simulink model "microgrid"  (R2025b)
settings: Solver=daessc  StartTime=0.0  StopTime=600  FixedStep=1728.0  MaxStep=1728.0  RelTol=1e-3
PreLoadFcn:
  | microgrid_parameters
InitFcn:
  | microgrid_parameters
values from neighbouring files (symbols this model uses):
  PV = photovoltaic_parameters    [microgrid_parameters.m]
  URFC = urfc_parameters    [microgrid_parameters.m]
undefined symbols (not defined in the file or in its folder): BUS, URFC_TANK
libraries: fl_lib x28, nesl_utility x14, ee_lib x9, SignalEditorBlockLib x1
settings Model: Creator=michaelfsb  LastModifiedBy=DEVANG
settings DebuggingCC: IgnoredZcDiagnostic=error
settings RTWCC: GPUComputeCapability=3.5
settings SimscapeCC: SimscapeLogLimitData=off

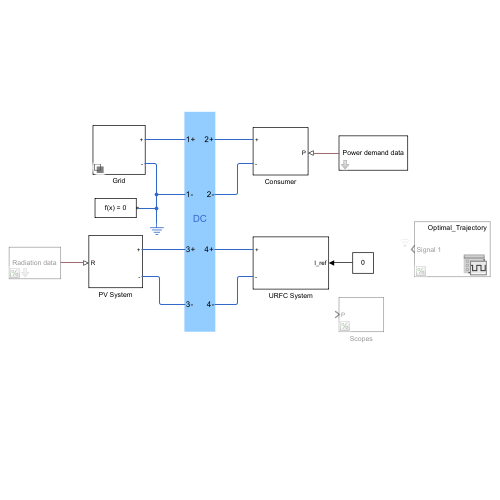
[thumbnail: Simulink's stored preview of the top-level diagram]
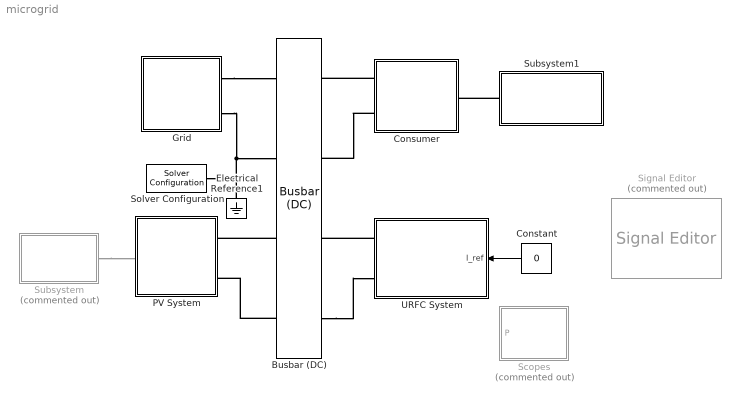
== system microgrid ==
  Busbar (DC) : ee_lib/Connectors & References/Busbar (DC)  n_nodes=ee.enum.connectors.busbar_number_of_connections.four  VRated=1e3 V  measurement_type=ee.enum.measurementType.instantaneous  averaging_period=1e-2 s  show_ps=ee.enum.connectors.busbar_measurement.false
      settings: InternalSimscapePortConfiguration="{\"Bottom\":[],\"Left\":[{\"id\":\"p1\",\"label\":\"1+\",\"type\":\"foundation.electrical.electrical\"},{\"id\":\"n1\",\"label\":\"1-\",\"type\":\"foundation.electrical.electrical\"},{\"id\":\"p3\",\"label\":\"3+\",\"type\":\"foundation.electrical.electrical\"},{\"id\":\"n3\",\"label\":\"3-\",\"type\":\"foundation.electrical.electrical\"}],\"Right\":[{\"id\":\"p2\",\"label\":\"2+\",\"type\":\"foundation.electrical.electrical\"},{\"id\":\"n2\",\"label\":\"2-\",\"type\":\"foundation.electrical.electrical\"},{\"id\":\"p4\",\"label\":\"4+\",\"type\":\"foundation.electrical.electrical\"},{\"id\":\"n4\",\"label\":\"4-\",\"type\":\"foundation.electrical.electrical\"}],\"Top\":[]}"
  Constant : Constant  Value=0
  Consumer : Subsystem
  Electrical Reference1 : fl_lib/Electrical/Electrical Elements/Electrical Reference
  Grid : Subsystem  Variant=on  VariantControlMode=label  VariantControl=Grid  LabelModeActiveChoice=AC1
      settings: PortSchema="{\"entries\":[{\"content\":{\"sides\":[{\"content\":{},\"type\":\"ConnectorPlacement.EquallySpacedRectSide\",\"uuid\":\"7d3e1531-3ac3-48d1-8d53-8dc071a39518\"},{\"content\":{\"side\":\"RIGHT\"},\"type\":\"ConnectorPlacement.EquallySpacedRectSide\",\"uuid\":\"25b50bd9-2b9f-4527-8fc7-8205feed0a4d\"},{\"content\":{\"connectorIds\":[\"LConn1\",\"LConn2\"],\"side\":\"TOP\"},\"type\":\"ConnectorPlacement.EquallySpacedRectSide\",\"uuid\":\"ec9d499b-92d3-45f6-91a8-3c7a2a7323b8\"}]},\"type\":\"ConnectorPlacement.EquallySpacedConnector\",\"uuid\":\"21f9d016-eefb-40e7-aeda-3b0d2900fe93\"}],\"packageUris\":[\"http://schema.mathworks.com/mf0/Connector/R2020b\"],\"version\":\"1.0\"}"
  PV System : Subsystem
      settings: PortSchema="{\"entries\":[{\"content\":{\"sides\":[{\"content\":{},\"type\":\"ConnectorPlacement.EquallySpacedRectSide\",\"uuid\":\"b223c642-574d-498e-9628-4dce2dfe786d\"},{\"content\":{\"side\":\"RIGHT\"},\"type\":\"ConnectorPlacement.EquallySpacedRectSide\",\"uuid\":\"c960ad2e-8659-4c85-9aee-0bfb29cbdae9\"},{\"content\":{\"connectorIds\":[\"LConn1\",\"LConn2\"],\"side\":\"TOP\"},\"type\":\"ConnectorPlacement.EquallySpacedRectSide\",\"uuid\":\"3aea4236-f32b-4c02-92e6-11ca7609eeb0\"},{\"content\":{\"connectorIds\":[\"RConn1\"],\"side\":\"BOTTOM\"},\"type\":\"ConnectorPlacement.EquallySpacedRectSide\",\"uuid\":\"59a771e4-e218-45af-8738-bea5dfc08a6d\"}]},\"type\":\"ConnectorPlacement.EquallySpacedConnector\",\"uuid\":\"f3a4f2e2-ab14-400c-a1b0-7ee7894a4fc3\"}],\"packageUris\":[\"http://schema.mathworks.com/mf0/Connector/R2020b\"],\"version\":\"1.0\"}"
  Scopes : Subsystem  Commented=on
  Signal Editor : SignalEditorBlockLib/Signal Editor  Commented=on  FileName=op_mode_siginal.mat  ActiveScenario=Optimal_Trajectory  ActiveSignal=i_el_ref  IsBus=off  OutputBusObjectStr=Bus: BusObject  SampleTime=0  ZeroCross=off  OutputAfterFinalValue=Setting to zero  Unit=inherit  PreserveSignalName=on  ApplySigPropsToAllScenarios=off  ApplySigPropsToAllSignals=on  SignalPropertySource=Dialog parameters
  Solver Configuration : nesl_utility/Solver Configuration  PhysicalDomain=network_engine_domain  SubClassName=solver  LeftPortType=input  RightPortType=generic  Tones=[]  Harmonics=[]  SimulateNoise=off  Profile=off  UseLocalSampling=off  EnableSwitchedLinearOptims=on  FrequencyDomain=off  UseCCode=off  RelTol=0.001  AbsTol=0.001  MinStep=1e-09  ToWorkspace=off  RevertToSquareIcSolve=off  NumHomotopyIterations=100  PhasorMode=off  PhasorModeNumHarmonics=1  ConsistencySolver=NEWTON_XTOL_AFTER_FTOL  IndexReductionMethod=DerivativeReplacement  DoDC=off  ResidualTolerance=1e-09  ConsistencyTolSource=GLOBAL  ConsistencyAbsTol=0.001  ConsistencyRelTol=0.001  ConsistencyTolFactor=0.001  UseLocalSolver=on  LocalSolverChoice=NE_BACKWARD_EULER_ADVANCER  ResolveIndetEquations=on  FunctionEvalNumThread=1  LocalSolverSampleTime=1  DoFixedCost=on  MaxNonlinIter=3  MaxModeIter=2  ComputeImpulses=off  ImpulseIterations=2  LinearAlgebra=auto  LinearAlgebraNumThread=0  EquationFormulation=NE_TIME_EF  DelaysMemoryBudget=1024  AutomaticFiltering=on  FilteringTimeConstant=0.001  PartitionStorageMethod=AS_NEEDED  PartitionMemoryBudget=1024  PartitionMethod=ROBUST  MultibodyUseLocalSolver=off  MultibodyLocalSolverChoice=ODE1  MultibodyLocalSolverSampleTime=0.001
  Subsystem : Subsystem  Commented=on
      mask Display: disp('Radiation data');
  Subsystem1 : Subsystem
      mask Display: disp('Power demand data');
  URFC System : Subsystem
  wires:
  Constant/1 -> URFC System/1(I_ref)
  connections:
  Busbar (DC)/LConn3 -- PV System/LConn1
  Consumer/LConn1 -- Busbar (DC)/RConn1
  Busbar (DC)/LConn4 -- PV System/LConn2
  Consumer/LConn2 -- Busbar (DC)/RConn2
  URFC System/RConn1 -- Busbar (DC)/RConn3
  Busbar (DC)/RConn4 -- URFC System/RConn2
  Subsystem/RConn1 -- PV System/RConn1
  Subsystem1/RConn1 -- Consumer/RConn1
  Grid/LConn2 -- Solver Configuration/RConn1 -- Electrical Reference1/LConn1 -- Busbar (DC)/LConn2
  Grid/LConn1 -- Busbar (DC)/LConn1

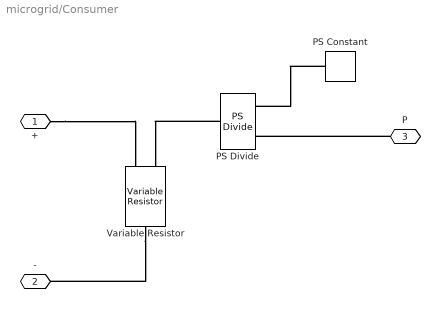
== system microgrid/Consumer ==
  PS Constant : fl_lib/Physical Signals/Sources/PS Constant  constant=BUS.Voltage^2 V^2
  PS Divide : fl_lib/Physical Signals/Functions/PS Divide
  Variable Resistor : fl_lib/Electrical/Electrical Elements/Variable Resistor  Rmin=0 Ohm  thermalEnable=false  thermal_mass=1 J/K  i_specify=off  i_priority=None  i=0 A  i_nominal_specify=off  i_nominal_value=1  i_nominal_unit=A  v_specify=off  v_priority=None  v=0 V  v_nominal_specify=off  v_nominal_value=1  v_nominal_unit=V  T_specify=off  T_priority=None  T=300 K  T_nominal_specify=off  T_nominal_value=1  T_nominal_unit=K
  + : PMIOPort  Side=Left
  - : PMIOPort  Port=2  Side=Left
  P : PMIOPort  Port=3  Side=Right
  connections:
  Variable Resistor/RConn1 -- -/RConn1
  PS Constant/RConn1 -- PS Divide/LConn1
  PS Divide/RConn1 -- Variable Resistor/LConn1
  +/RConn1 -- Variable Resistor/LConn2
  P/RConn1 -- PS Divide/LConn2

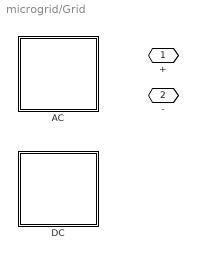
== system microgrid/Grid ==
  AC : Subsystem  VariantControl=Grid
      settings: PortSchema="{\"entries\":[{\"content\":{\"sides\":[{\"content\":{},\"type\":\"ConnectorPlacement.EquallySpacedRectSide\",\"uuid\":\"7d3e1531-3ac3-48d1-8d53-8dc071a39518\"},{\"content\":{\"side\":\"RIGHT\"},\"type\":\"ConnectorPlacement.EquallySpacedRectSide\",\"uuid\":\"25b50bd9-2b9f-4527-8fc7-8205feed0a4d\"},{\"content\":{\"connectorIds\":[\"LConn1\",\"LConn2\"],\"side\":\"TOP\"},\"type\":\"ConnectorPlacement.EquallySpacedRectSide\",\"uuid\":\"ec9d499b-92d3-45f6-91a8-3c7a2a7323b8\"}]},\"type\":\"ConnectorPlacement.EquallySpacedConnector\",\"uuid\":\"21f9d016-eefb-40e7-aeda-3b0d2900fe93\"}],\"packageUris\":[\"http://schema.mathworks.com/mf0/Connector/R2020b\"],\"version\":\"1.0\"}"
  DC : Subsystem  VariantControl=AC1
      settings: PortSchema="{\"entries\":[{\"content\":{\"sides\":[{\"content\":{},\"type\":\"ConnectorPlacement.EquallySpacedRectSide\",\"uuid\":\"7d3e1531-3ac3-48d1-8d53-8dc071a39518\"},{\"content\":{\"side\":\"RIGHT\"},\"type\":\"ConnectorPlacement.EquallySpacedRectSide\",\"uuid\":\"25b50bd9-2b9f-4527-8fc7-8205feed0a4d\"},{\"content\":{\"connectorIds\":[\"LConn1\",\"LConn2\"],\"side\":\"TOP\"},\"type\":\"ConnectorPlacement.EquallySpacedRectSide\",\"uuid\":\"ec9d499b-92d3-45f6-91a8-3c7a2a7323b8\"}]},\"type\":\"ConnectorPlacement.EquallySpacedConnector\",\"uuid\":\"21f9d016-eefb-40e7-aeda-3b0d2900fe93\"}],\"packageUris\":[\"http://schema.mathworks.com/mf0/Connector/R2020b\"],\"version\":\"1.0\"}"
  + : PMIOPort  Side=Left
  - : PMIOPort  Port=2  Side=Left

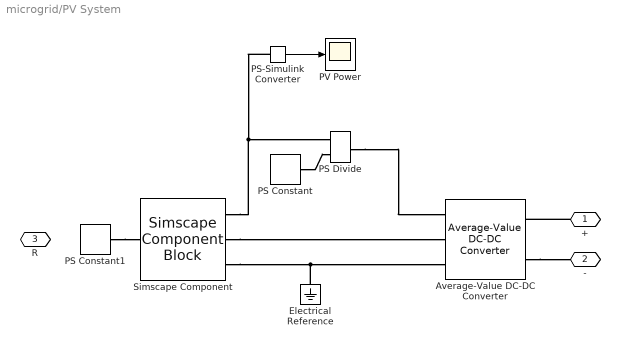
== system microgrid/PV System ==
  Average-Value DC-DC Converter : ee_lib/Semiconductors & Converters/Converters/Average-Value DC-DC Converter  implementation_option=ee.enum.converters.implementation.behavioral  converter_type=ee.enum.converters.dcdctype.boost  control_option=ee.enum.converters.controlinput.current  efficiency_option=ee.enum.converters.efficiency.constant  efficiency_fixed=100  i_vec=[0, 2, 5] A  efficiency_vec=[90, 95, 98]  Lf=1e-6 H  Rl=0 Ohm  Cf=1e-7 F  Rc=1e-6 Ohm  iL_specify=off  iL_priority=High  iL=0 A  iL_nominal_specify=off  iL_nominal_value=1  iL_nominal_unit=A  vc_specify=off  vc_priority=High  vc=0 V  vc_nominal_specify=off  vc_nominal_value=1  vc_nominal_unit=V
      settings: InternalSimscapePortConfiguration="{\"Bottom\":[],\"Left\":[{\"id\":\"Iref\",\"label\":\"Iref\",\"type\":\"input\"},{\"id\":\"p1\",\"label\":\"1+\",\"type\":\"foundation.electrical.electrical\"},{\"id\":\"n1\",\"label\":\"1-\",\"type\":\"foundation.electrical.electrical\"}],\"Right\":[{\"id\":\"p2\",\"label\":\"2+\",\"type\":\"foundation.electrical.electrical\"},{\"id\":\"n2\",\"label\":\"2-\",\"type\":\"foundation.electrical.electrical\"}],\"Top\":[]}"
  Electrical Reference : fl_lib/Electrical/Electrical Elements/Electrical Reference
  PS Constant : fl_lib/Physical Signals/Sources/PS Constant  constant=BUS.Voltage V
  PS Constant1 : fl_lib/Physical Signals/Sources/PS Constant  constant=0.5
  PS Divide : fl_lib/Physical Signals/Functions/PS Divide
  PS-Simulink Converter : nesl_utility/PS-Simulink Converter  PhysicalDomain=network_engine_domain  SubClassName=ps_output  LeftPortType=input  RightPortType=output  PseudoPeriodic=off  Frequencies=[]  VectorFormat=inherit  Unit=W  AffineConversion=off
  PV Power : Scope
      settings: ActiveDisplayYMinimum=2487.8736060654028  ActiveDisplayYMaximum=4487.8736060654028  DataLoggingVariableName=ScopeData4
  Simscape Component : SimscapeComponentBlock  SourceFile=pv_panel  ComponentPath=pv_panel  ComponentVariants="[\"pv_panel\"]"  ComponentVariantNames="[\"pv_panel\"]"  ClassName=pv_panel  SchemaVersion=1  Nps=PV.N_ps  Nss=PV.N_ss  T=PV.T_ps K  Tr=PV.Tr K  Isc=PV.Isc A  Kl=PV.Kl A/K  Ior=PV.Ior A  Ego=PV.Ego V  A=PV.A  v_specify=off  v_priority=None  v=0 V  v_nominal_specify=off  v_nominal_value=1  v_nominal_unit=V  i_specify=off  i_priority=None  i=0 A  i_nominal_specify=off  i_nominal_value=1  i_nominal_unit=A
      settings: CopyFcn=simscape.sscblock.internal.componentBlockCallback(gcbh,'COPY')  PreCopyFcn=simscape.sscblock.internal.componentBlockCallback(gcbh,'PRECOPY')  PreDeleteFcn=simscape.sscblock.internal.componentBlockCallback(gcbh,'PREDELETE')  InternalSimscapePortConfiguration="{\"Bottom\":[],\"Left\":[{\"id\":\"lambda\",\"label\":\"R\",\"type\":\"input\"}],\"Right\":[{\"id\":\"p_mppt\",\"label\":\"p\",\"type\":\"output\"},{\"id\":\"p\",\"label\":\"+\",\"type\":\"foundation.electrical.electrical\"},{\"id\":\"n\",\"label\":\"-\",\"type\":\"foundation.electrical.electrical\"}],\"Top\":[]}"
      mask Type: pv_panel
  + : PMIOPort  Side=Left
  - : PMIOPort  Port=2  Side=Left
  R : PMIOPort  Port=3  Side=Right
  wires:
  PS-Simulink Converter/1 -> PV Power/1
  connections:
  Electrical Reference/LConn1 -- Average-Value DC-DC Converter/LConn3 -- Simscape Component/RConn3
  Simscape Component/RConn2 -- Average-Value DC-DC Converter/LConn2
  PS Constant/RConn1 -- PS Divide/LConn2
  Simscape Component/RConn1 -- PS-Simulink Converter/LConn1 -- PS Divide/LConn1
  PS Divide/RConn1 -- Average-Value DC-DC Converter/LConn1
  +/RConn1 -- Average-Value DC-DC Converter/RConn1
  Average-Value DC-DC Converter/RConn2 -- -/RConn1
  PS Constant1/RConn1 -- Simscape Component/LConn1

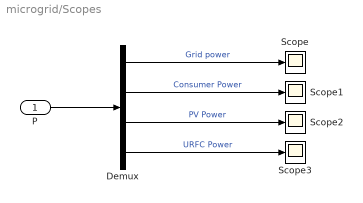
== system microgrid/Scopes ==
  P : Inport
  Demux : Demux
  Scope{,1..3} (4 alike) : Scope
      Scope2 settings: DataLoggingVariableName=ScopeData2
      Scope3 settings: DataLoggingVariableName=ScopeData3
  wires:
  P/1 -> Demux/1
  Demux/1 -> Scope/1  "Grid power"
  Demux/4 -> Scope3/1  "URFC Power"
  Demux/2 -> Scope1/1  "Consumer Power"
  Demux/3 -> Scope2/1  "PV Power"

== system microgrid/Subsystem ==
  PS Lookup Table (1D) : fl_lib/Physical Signals/Lookup Tables/PS Lookup Table (1D)  x=radiation.time  f=radiation.data  interp_method=simscape.enum.interpolation.linear  extrap_method=simscape.enum.extrapolation.linear
  PS Ramp : fl_lib/Physical Signals/Sources/PS Ramp  slope=1 1/s  start_time=0 s  initial_output=0  ZeroCross=true
  Conn1 : PMIOPort  Side=Right
  connections:
  PS Lookup Table (1D)/RConn1 -- Conn1/RConn1
  PS Ramp/RConn1 -- PS Lookup Table (1D)/LConn1

== system microgrid/Subsystem1 ==
  PS Lookup Table (1D)1 : fl_lib/Physical Signals/Lookup Tables/PS Lookup Table (1D)  x=power_demand.time  f=power_demand.data W  interp_method=simscape.enum.interpolation.linear  extrap_method=simscape.enum.extrapolation.linear
  PS Ramp1 : fl_lib/Physical Signals/Sources/PS Ramp  slope=1 1/s  start_time=0 s  initial_output=0  ZeroCross=true
  Conn1 : PMIOPort  Side=Right
  connections:
  PS Lookup Table (1D)1/RConn1 -- Conn1/RConn1
  PS Ramp1/RConn1 -- PS Lookup Table (1D)1/LConn1

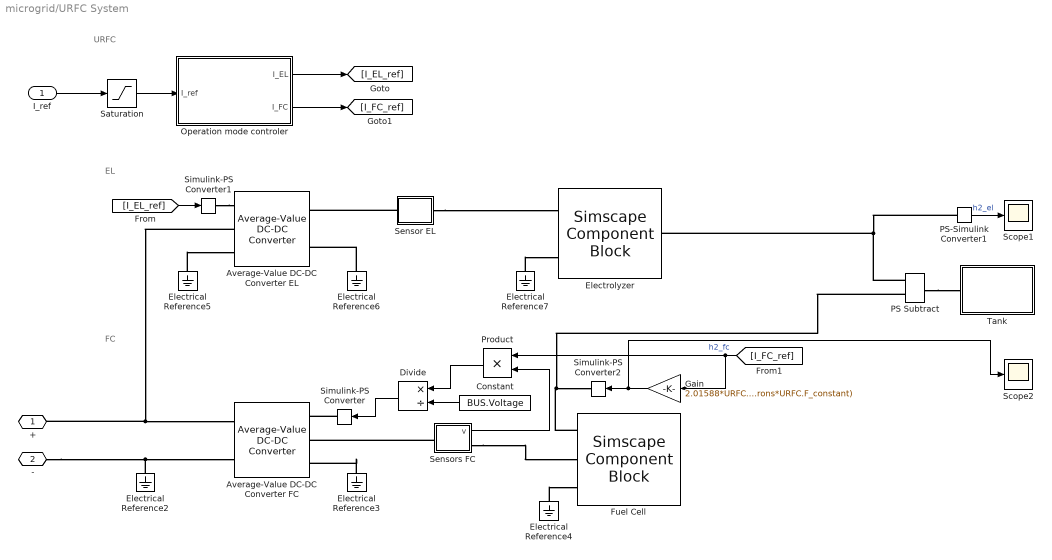
== system microgrid/URFC System ==
  note: URFC
  note: FC
  note: EL
  I_ref : Inport
  Average-Value DC-DC Converter EL : ee_lib/Semiconductors & Converters/Converters/Average-Value DC-DC Converter  implementation_option=ee.enum.converters.implementation.behavioral  converter_type=ee.enum.converters.dcdctype.buck  control_option=ee.enum.converters.controlinput.current  efficiency_option=ee.enum.converters.efficiency.tabulated  efficiency_fixed=100  i_vec=[0, 100, 200] A  efficiency_vec=[90, 95, 98]  Lf=1e-6 H  Rl=0 Ohm  Cf=1e-7 F  Rc=1e-6 Ohm  iL_specify=off  iL_priority=High  iL=0 A  iL_nominal_specify=off  iL_nominal_value=1  iL_nominal_unit=A  vc_specify=off  vc_priority=High  vc=0 V  vc_nominal_specify=off  vc_nominal_value=1  vc_nominal_unit=V
      settings: InternalSimscapePortConfiguration="{\"Bottom\":[],\"Left\":[{\"id\":\"Iref\",\"label\":\"Iref\",\"type\":\"input\"},{\"id\":\"p1\",\"label\":\"1+\",\"type\":\"foundation.electrical.electrical\"},{\"id\":\"n1\",\"label\":\"1-\",\"type\":\"foundation.electrical.electrical\"}],\"Right\":[{\"id\":\"p2\",\"label\":\"2+\",\"type\":\"foundation.electrical.electrical\"},{\"id\":\"n2\",\"label\":\"2-\",\"type\":\"foundation.electrical.electrical\"}],\"Top\":[]}"
  Average-Value DC-DC Converter FC : ee_lib/Semiconductors & Converters/Converters/Average-Value DC-DC Converter  implementation_option=ee.enum.converters.implementation.behavioral  converter_type=ee.enum.converters.dcdctype.boost  control_option=ee.enum.converters.controlinput.current  efficiency_option=ee.enum.converters.efficiency.constant  efficiency_fixed=100  i_vec=[0, 0.75, 2] A  efficiency_vec=[90, 95, 98]  Lf=1e-6 H  Rl=0 Ohm  Cf=1e-7 F  Rc=1e-6 Ohm  iL_specify=off  iL_priority=High  iL=0 A  iL_nominal_specify=off  iL_nominal_value=1  iL_nominal_unit=A  vc_specify=off  vc_priority=High  vc=0 V  vc_nominal_specify=off  vc_nominal_value=1  vc_nominal_unit=V
      settings: InternalSimscapePortConfiguration="{\"Bottom\":[],\"Left\":[{\"id\":\"Iref\",\"label\":\"Iref\",\"type\":\"input\"},{\"id\":\"p1\",\"label\":\"1+\",\"type\":\"foundation.electrical.electrical\"},{\"id\":\"n1\",\"label\":\"1-\",\"type\":\"foundation.electrical.electrical\"}],\"Right\":[{\"id\":\"p2\",\"label\":\"2+\",\"type\":\"foundation.electrical.electrical\"},{\"id\":\"n2\",\"label\":\"2-\",\"type\":\"foundation.electrical.electrical\"}],\"Top\":[]}"
  Constant : Constant  Value=BUS.Voltage
  Divide : Product  Inputs=*/
  Electrical Reference{2..7} (6 alike) : fl_lib/Electrical/Electrical Elements/Electrical Reference
  Electrolyzer : SimscapeComponentBlock  SourceFile=urfc_electrolyzer  ComponentPath=urfc_electrolyzer  ComponentVariants="[\"urfc_electrolyzer\"]"  ComponentVariantNames="[\"urfc_electrolyzer\"]"  ClassName=urfc_electrolyzer  SchemaVersion=1  N_cells=URFC.N_cells  A_cell=URFC.A_cell cm^2  E_rev_0=URFC.E_rev_0 V  I_loss_internal=URFC.I_loss_internal A/cm^2  I_o_anode=URFC.I_o_anode A/cm^2  I_o_cathode=URFC.I_o_cathode A/cm^2  R_ion=URFC.R_ion Ohm*cm^2  R_CR=URFC.R_CR Ohm*cm^2  R_elect=URFC.R_elect Ohm*cm^2  I_limit_anode=URFC.I_limit_anode A/cm^2  I_limit_cathode=URFC.I_limit_cathode A/cm^2  A_anodo=URFC.K_anodo V  A_catodo=URFC.K_catodo V  T=URFC.T K  R_gas=URFC.R_gas J/(K*mol)  F_constant=URFC.F_constant C/mol  n_electrons=URFC.n_electrons  i_specify=off  i_priority=None  i=0 A  i_nominal_specify=off  i_nominal_value=1  i_nominal_unit=A  v_specify=off  v_priority=None  v=0 V  v_nominal_specify=off  v_nominal_value=1  v_nominal_unit=V
      settings: CopyFcn=simscape.sscblock.internal.componentBlockCallback(gcbh,'COPY')  PreCopyFcn=simscape.sscblock.internal.componentBlockCallback(gcbh,'PRECOPY')  PreDeleteFcn=simscape.sscblock.internal.componentBlockCallback(gcbh,'PREDELETE')  LogSimulationData=on  InternalSimscapePortConfiguration="{\"Bottom\":[],\"Left\":[{\"id\":\"p\",\"label\":\"+\",\"type\":\"foundation.electrical.electrical\"},{\"id\":\"n\",\"label\":\"-\",\"type\":\"foundation.electrical.electrical\"}],\"Right\":[{\"id\":\"h2\",\"label\":\"H2\",\"type\":\"output\"}],\"Top\":[]}"
      mask Type: Electrolyzer mode model of a URFC
  Fuel Cell : SimscapeComponentBlock  SourceFile=urfc_fuel_cell  ComponentPath=urfc_fuel_cell  ComponentVariants="[\"urfc_fuel_cell\"]"  ComponentVariantNames="[\"urfc_fuel_cell\"]"  ClassName=urfc_fuel_cell  SchemaVersion=1  N_cells=URFC.N_cells  A_cell=URFC.A_cell cm^2  E_rev_0=1.23 V  I_loss_internal=URFC.I_loss_internal A/cm^2  I_o_anode=URFC.I_o_anode A/cm^2  I_o_cathode=URFC.I_o_cathode A/cm^2  R_ion=URFC.R_ion Ohm*cm^2  R_CR=URFC.R_CR Ohm*cm^2  R_elect=URFC.R_elect Ohm*cm^2  I_limit_anode=URFC.I_limit_anode A/cm^2  I_limit_cathode=URFC.I_limit_cathode A/cm^2  A_anodo=URFC.K_anodo V  A_catodo=URFC.K_catodo V  T=URFC.T K  R_gas=URFC.R_gas J/(K*mol)  F_constant=URFC.F_constant C/mol  n_electrons=2  i_specify=off  i_priority=None  i=0 A  i_nominal_specify=off  i_nominal_value=1  i_nominal_unit=A  v_specify=off  v_priority=None  v=0 V  v_nominal_specify=off  v_nominal_value=1  v_nominal_unit=V
      settings: CopyFcn=simscape.sscblock.internal.componentBlockCallback(gcbh,'COPY')  PreCopyFcn=simscape.sscblock.internal.componentBlockCallback(gcbh,'PRECOPY')  PreDeleteFcn=simscape.sscblock.internal.componentBlockCallback(gcbh,'PREDELETE')  LogSimulationData=on  InternalSimscapePortConfiguration="{\"Bottom\":[],\"Left\":[{\"id\":\"h2_in\",\"label\":\"H2_in\",\"type\":\"input\"},{\"id\":\"p\",\"label\":\"+\",\"type\":\"foundation.electrical.electrical\"},{\"id\":\"n\",\"label\":\"-\",\"type\":\"foundation.electrical.electrical\"}],\"Right\":[],\"Top\":[]}"
      mask Type: Fuel Cell mode model of a URFC
  Gain : Gain  Gain=2.01588*URFC.N_cells/(URFC.n_electrons*URFC.F_constant)
  Operation mode controler : Stateflow chart  TreatAsAtomicUnit=on
  PS Subtract : fl_lib/Physical Signals/Functions/PS Subtract
  PS-Simulink Converter1 : nesl_utility/PS-Simulink Converter  PhysicalDomain=network_engine_domain  SubClassName=ps_output  LeftPortType=input  RightPortType=output  PseudoPeriodic=off  Frequencies=[]  VectorFormat=inherit  Unit=inherit  AffineConversion=off
  Product : Product
  Saturation : Saturate  UpperLimit=200  LowerLimit=-200
  Scope1 : Scope
      settings: ActiveDisplayYMinimum=-0.00418  ActiveDisplayYMaximum=0.03763
  Scope2 : Scope
      settings: ActiveDisplayYMinimum=-1  ActiveDisplayYMaximum=1  DataLoggingVariableName=ScopeData2
  Sensor EL : Subsystem
  Sensors FC : Subsystem
  Simulink-PS Converter : nesl_utility/Simulink-PS Converter  PhysicalDomain=network_engine_domain  SubClassName=ps_input  LeftPortType=input  RightPortType=output  PseudoPeriodic=off  Frequencies=[]  NoiseDistribution=none  NoiseParameters=[]  Unit=1  AffineConversion=off  FilteringAndDerivatives=provide  SimscapeFilterOrder=1  InputFilterTimeConstant=0.001  UdotUserProvided=0
  Simulink-PS Converter1 : nesl_utility/Simulink-PS Converter  PhysicalDomain=network_engine_domain  SubClassName=ps_input  LeftPortType=input  RightPortType=output  PseudoPeriodic=off  Frequencies=[]  NoiseDistribution=none  NoiseParameters=[]  Unit=1  AffineConversion=off  FilteringAndDerivatives=provide  SimscapeFilterOrder=1  InputFilterTimeConstant=0.001  UdotUserProvided=0
  Simulink-PS Converter2 : nesl_utility/Simulink-PS Converter  PhysicalDomain=network_engine_domain  SubClassName=ps_input  LeftPortType=input  RightPortType=output  PseudoPeriodic=off  Frequencies=[]  NoiseDistribution=none  NoiseParameters=[]  Unit=g/s  AffineConversion=off  FilteringAndDerivatives=provide  SimscapeFilterOrder=1  InputFilterTimeConstant=0.001  UdotUserProvided=0
  Tank : Subsystem
  + : PMIOPort  Side=Right
  - : PMIOPort  Port=2  Side=Right
  wires:
  Constant/1 -> Divide/2
  Product/1 -> Divide/1
  [I_FC_ref] -> Gain/1, Product/1
  Sensors FC/1(v) -> Product/2
  Divide/1 -> Simulink-PS Converter/1
  Saturation/1 -> Operation mode controler/1(I_ref)
  Operation mode controler/2(I_FC) -> [I_FC_ref]
  Operation mode controler/1(I_EL) -> [I_EL_ref]
  I_ref/1 -> Saturation/1
  [I_EL_ref] -> Simulink-PS Converter1/1
  Gain/1 -> Scope2/1, Simulink-PS Converter2/1  "h2_fc"
  PS-Simulink Converter1/1 -> Scope1/1  "h2_el"
  connections:
  Sensors FC/RConn1 -- Fuel Cell/LConn2
  PS-Simulink Converter1/LConn1 -- PS Subtract/LConn1 -- Electrolyzer/RConn1
  Electrical Reference5/LConn1 -- Average-Value DC-DC Converter EL/LConn3
  Simulink-PS Converter1/RConn1 -- Average-Value DC-DC Converter EL/LConn1
  Electrical Reference6/LConn1 -- Average-Value DC-DC Converter EL/RConn2
  Sensor EL/RConn1 -- Average-Value DC-DC Converter EL/RConn1
  Sensors FC/LConn1 -- Average-Value DC-DC Converter FC/LConn2
  Simulink-PS Converter/RConn1 -- Average-Value DC-DC Converter FC/LConn1
  Electrical Reference3/LConn1 -- Average-Value DC-DC Converter FC/LConn3
  Electrical Reference2/LConn1 -- -/RConn1 -- Average-Value DC-DC Converter FC/RConn2
  Average-Value DC-DC Converter EL/LConn2 -- +/RConn1 -- Average-Value DC-DC Converter FC/RConn1
  Electrical Reference4/LConn1 -- Fuel Cell/LConn3
  Sensor EL/LConn1 -- Electrolyzer/LConn1
  Electrical Reference7/LConn1 -- Electrolyzer/LConn2
  PS Subtract/RConn1 -- Tank/LConn1
  Fuel Cell/LConn1 -- PS Subtract/LConn2 -- Simulink-PS Converter2/RConn1

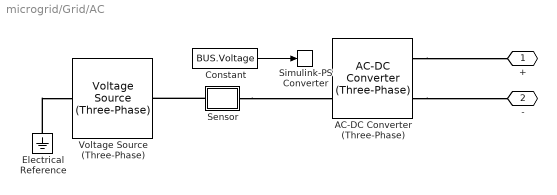
== system microgrid/Grid/AC ==
  AC-DC Converter (Three-Phase) : ee_lib/Semiconductors & Converters/Converters/AC-DC Converter (Three-Phase)  port_option=ee.enum.threePhasePort.composite  droop=0 V/A  Vdc_dynamics=ee.enum.converters.dynamics.no  tauVdc=0.02 s  Vdc_ini=100 V  FRated=60 Hz  Vline_rms_min=0.8*sqrt(3) * 100 / sqrt(2) V  tauVac=0.001 s  Vline_rms_ini=sqrt(3) * 100 / sqrt(2) V  Vang_ini=0 deg  power_dynamics=ee.enum.converters.powerDynamics.no  tauP=0.01 s  P_ini=1e3 W  gmin=1e-6 S
      settings: InternalSimscapePortConfiguration="{\"Bottom\":[],\"Left\":[{\"id\":\"Vref\",\"label\":\"Vref\",\"type\":\"input\"},{\"id\":\"N\",\"label\":\"~\",\"type\":\"foundation.electrical.three_phase\"}],\"Right\":[{\"id\":\"p\",\"label\":\"+\",\"type\":\"foundation.electrical.electrical\"},{\"id\":\"n\",\"label\":\"-\",\"type\":\"foundation.electrical.electrical\"}],\"Top\":[]}"
  Constant : Constant  Value=BUS.Voltage
  Electrical Reference : fl_lib/Electrical/Electrical Elements/Electrical Reference
  Sensor : Subsystem
      mask Display: disp('P');
  Simulink-PS Converter : nesl_utility/Simulink-PS Converter  PhysicalDomain=network_engine_domain  SubClassName=ps_input  LeftPortType=input  RightPortType=output  PseudoPeriodic=off  Frequencies=[]  NoiseDistribution=none  NoiseParameters=[]  Unit=V  AffineConversion=off  FilteringAndDerivatives=provide  SimscapeFilterOrder=1  InputFilterTimeConstant=0.001  UdotUserProvided=0
  Voltage Source (Three-Phase) : ee_lib/Sources/Voltage Source (Three-Phase)  vline_rms=sqrt(3) * 100 / sqrt(2) V  shift=0 deg  freq=60 Hz  impedance_option=1  SShortCircuit=1e6 A*V  XR=15  R=0.01 Ohm  L=3.97e-4 H  harmonic_option=0  harmonic_orders=[5, 7, 11, 13]  harmonic_ratios=[.1, .1, .1, .1]  G_parasitic=0 1/Ohm  I_specify=off  I_priority=None  I=[0, 0, 0] A  I_nominal_specify=off  I_nominal_unit=A  I_nominal_value=1
  + : PMIOPort  Side=Left
  - : PMIOPort  Port=2  Side=Left
  wires:
  Constant/1 -> Simulink-PS Converter/1
  connections:
  AC-DC Converter (Three-Phase)/RConn1 -- +/RConn1
  AC-DC Converter (Three-Phase)/RConn2 -- -/RConn1
  Sensor/RConn1 -- AC-DC Converter (Three-Phase)/LConn2
  Sensor/LConn1 -- Voltage Source (Three-Phase)/RConn1
  Electrical Reference/LConn1 -- Voltage Source (Three-Phase)/LConn1

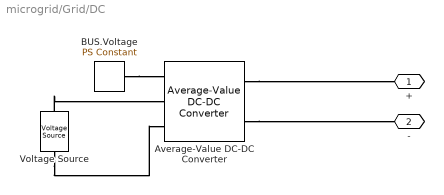
== system microgrid/Grid/DC ==
  Average-Value DC-DC Converter : ee_lib/Semiconductors & Converters/Converters/Average-Value DC-DC Converter  implementation_option=ee.enum.converters.implementation.behavioral  converter_type=ee.enum.converters.dcdctype.buck  control_option=ee.enum.converters.controlinput.voltage  efficiency_option=ee.enum.converters.efficiency.constant  efficiency_fixed=95  i_vec=[0, 2, 5] A  efficiency_vec=[90, 95, 98]  Lf=1e-6 H  Rl=0 Ohm  Cf=1e-7 F  Rc=1e-6 Ohm  iL_specify=off  iL_priority=High  iL=0 A  iL_nominal_specify=off  iL_nominal_value=1  iL_nominal_unit=A  vc_specify=off  vc_priority=High  vc=0 V  vc_nominal_specify=off  vc_nominal_value=1  vc_nominal_unit=V
      settings: InternalSimscapePortConfiguration="{\"Bottom\":[],\"Left\":[{\"id\":\"Vref\",\"label\":\"Vref\",\"type\":\"input\"},{\"id\":\"p1\",\"label\":\"1+\",\"type\":\"foundation.electrical.electrical\"},{\"id\":\"n1\",\"label\":\"1-\",\"type\":\"foundation.electrical.electrical\"}],\"Right\":[{\"id\":\"p2\",\"label\":\"2+\",\"type\":\"foundation.electrical.electrical\"},{\"id\":\"n2\",\"label\":\"2-\",\"type\":\"foundation.electrical.electrical\"}],\"Top\":[]}"
  BUS.Voltage : fl_lib/Physical Signals/Sources/PS Constant  constant=BUS.Voltage V
  Voltage Source : ee_lib/Sources/Voltage Source  dc_voltage=BUS.Voltage V  ac_voltage=0 V  ac_shift=0 rad  ac_frequency=60 Hz  noise_mode=ee.enum.sources.noise.Disabled  PSD=0 V^2/Hz  sample_time=1e-3 s  repeatability=ee.enum.sources.repeatability.NotRepeatable  user_seed=0  auto_seed=1129453067  i_specify=off  i_priority=None  i=0 A  i_nominal_specify=off  i_nominal_value=1  i_nominal_unit=A  v_specify=off  v_priority=None  v=0 V  v_nominal_specify=off  v_nominal_value=1  v_nominal_unit=V
  + : PMIOPort  Side=Left
  - : PMIOPort  Port=2  Side=Left
  connections:
  Voltage Source/LConn1 -- Average-Value DC-DC Converter/LConn2
  Voltage Source/RConn1 -- Average-Value DC-DC Converter/LConn3
  BUS.Voltage/RConn1 -- Average-Value DC-DC Converter/LConn1
  Average-Value DC-DC Converter/RConn1 -- +/RConn1
  Average-Value DC-DC Converter/RConn2 -- -/RConn1

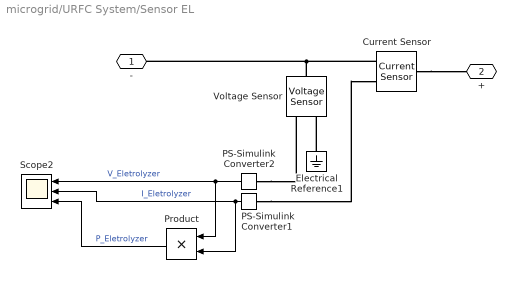
== system microgrid/URFC System/Sensor EL ==
  Current Sensor : fl_lib/Electrical/Electrical Sensors/Current Sensor
  Electrical Reference1 : fl_lib/Electrical/Electrical Elements/Electrical Reference
  PS-Simulink Converter1 : nesl_utility/PS-Simulink Converter  PhysicalDomain=network_engine_domain  SubClassName=ps_output  LeftPortType=input  RightPortType=output  PseudoPeriodic=off  Frequencies=[]  VectorFormat=inherit  Unit=inherit  AffineConversion=off
  PS-Simulink Converter2 : nesl_utility/PS-Simulink Converter  PhysicalDomain=network_engine_domain  SubClassName=ps_output  LeftPortType=input  RightPortType=output  PseudoPeriodic=off  Frequencies=[]  VectorFormat=inherit  Unit=inherit  AffineConversion=off
  Product : Product
  Scope2 : Scope  NumInputPorts=3
      settings: ActiveDisplayYMinimum=-52.2579  ActiveDisplayYMaximum=561.36199
  Voltage Sensor : fl_lib/Electrical/Electrical Sensors/Voltage Sensor
  - : PMIOPort  Side=Left
  + : PMIOPort  Port=2  Side=Right
  wires:
  PS-Simulink Converter2/1 -> Product/1, Scope2/1  "V_Eletrolyzer"
  PS-Simulink Converter1/1 -> Scope2/2, Product/2  "I_Eletrolyzer"
  Product/1 -> Scope2/3  "P_Eletrolyzer"
  connections:
  Current Sensor/LConn1 -- +/RConn1
  Electrical Reference1/LConn1 -- Voltage Sensor/RConn2
  PS-Simulink Converter2/LConn1 -- Voltage Sensor/RConn1
  Current Sensor/RConn2 -- Voltage Sensor/LConn1 -- -/RConn1
  PS-Simulink Converter1/LConn1 -- Current Sensor/RConn1

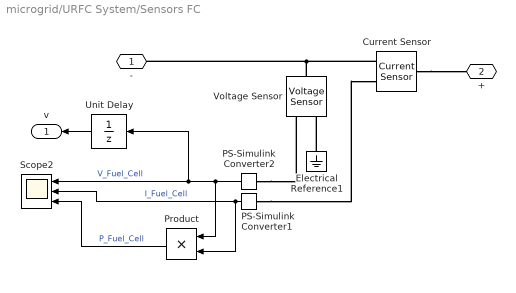
== system microgrid/URFC System/Sensors FC ==
  Current Sensor : fl_lib/Electrical/Electrical Sensors/Current Sensor
  Electrical Reference1 : fl_lib/Electrical/Electrical Elements/Electrical Reference
  PS-Simulink Converter1 : nesl_utility/PS-Simulink Converter  PhysicalDomain=network_engine_domain  SubClassName=ps_output  LeftPortType=input  RightPortType=output  PseudoPeriodic=off  Frequencies=[]  VectorFormat=inherit  Unit=inherit  AffineConversion=off
  PS-Simulink Converter2 : nesl_utility/PS-Simulink Converter  PhysicalDomain=network_engine_domain  SubClassName=ps_output  LeftPortType=input  RightPortType=output  PseudoPeriodic=off  Frequencies=[]  VectorFormat=inherit  Unit=inherit  AffineConversion=off
  Product : Product
  Scope2 : Scope  NumInputPorts=3
      settings: ActiveDisplayYMinimum=-52.2579  ActiveDisplayYMaximum=561.36199
  Unit Delay : UnitDelay  SampleTime=-1  HasFrameUpgradeWarning=on
  Voltage Sensor : fl_lib/Electrical/Electrical Sensors/Voltage Sensor
  - : PMIOPort  Side=Left
  + : PMIOPort  Port=2  Side=Right
  v : Outport
  wires:
  PS-Simulink Converter2/1 -> Product/1, Unit Delay/1, Scope2/1  "V_Fuel_Cell"
  PS-Simulink Converter1/1 -> Scope2/2, Product/2  "I_Fuel_Cell"
  Product/1 -> Scope2/3  "P_Fuel_Cell"
  Unit Delay/1 -> v/1
  connections:
  Current Sensor/LConn1 -- +/RConn1
  Electrical Reference1/LConn1 -- Voltage Sensor/RConn2
  PS-Simulink Converter2/LConn1 -- Voltage Sensor/RConn1
  Current Sensor/RConn2 -- -/RConn1 -- Voltage Sensor/LConn1
  PS-Simulink Converter1/LConn1 -- Current Sensor/RConn1

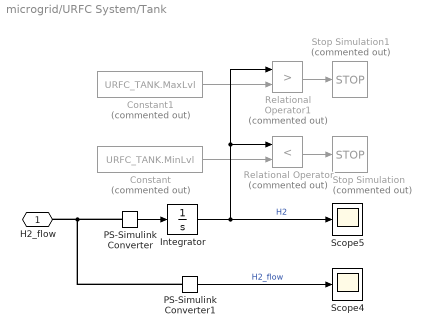
== system microgrid/URFC System/Tank ==
  Constant : Constant  Commented=on  Value=URFC_TANK.MinLvl
  Constant1 : Constant  Commented=on  Value=URFC_TANK.MaxLvl
  Integrator : Integrator  InitialCondition=URFC_TANK.IniLvl  AbsoluteTolerance=-1
  PS-Simulink Converter : nesl_utility/PS-Simulink Converter  PhysicalDomain=network_engine_domain  SubClassName=ps_output  LeftPortType=input  RightPortType=output  PseudoPeriodic=off  Frequencies=[]  VectorFormat=inherit  Unit=inherit  AffineConversion=off
  PS-Simulink Converter1 : nesl_utility/PS-Simulink Converter  PhysicalDomain=network_engine_domain  SubClassName=ps_output  LeftPortType=input  RightPortType=output  PseudoPeriodic=off  Frequencies=[]  VectorFormat=inherit  Unit=inherit  AffineConversion=off
  Relational Operator : RelationalOperator  Commented=on  Operator=<  OutDataTypeStr=boolean  RndMeth=Simplest  InputSameDT=off
  Relational Operator1 : RelationalOperator  Commented=on  Operator=>  OutDataTypeStr=boolean  RndMeth=Simplest  InputSameDT=off
  Scope4 : Scope
      settings: ActiveDisplayYMinimum=-0.02622  ActiveDisplayYMaximum=-0.00622  DataLoggingVariableName=ScopeData3
  Scope5 : Scope
      settings: ActiveDisplayYMinimum=-1  ActiveDisplayYMaximum=1
  Stop Simulation : Stop  Commented=on
  Stop Simulation1 : Stop  Commented=on
  H2_flow : PMIOPort  Side=Left
  wires:
  PS-Simulink Converter1/1 -> Scope4/1  "H2_flow"
  Constant/1 -> Relational Operator/2
  Relational Operator/1 -> Stop Simulation/1
  PS-Simulink Converter/1 -> Integrator/1
  Constant1/1 -> Relational Operator1/2
  Relational Operator1/1 -> Stop Simulation1/1
  Integrator/1 -> Relational Operator1/1, Relational Operator/1, Scope5/1  "H2"
  connections:
  PS-Simulink Converter1/LConn1 -- PS-Simulink Converter/LConn1 -- H2_flow/RConn1

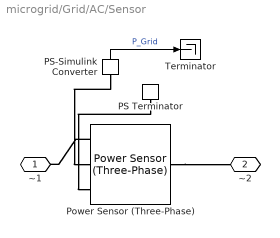
== system microgrid/Grid/AC/Sensor ==
  PS Terminator : fl_lib/Physical Signals/Sinks/PS Terminator
  PS-Simulink Converter : nesl_utility/PS-Simulink Converter  PhysicalDomain=network_engine_domain  SubClassName=ps_output  LeftPortType=input  RightPortType=output  PseudoPeriodic=off  Frequencies=[]  VectorFormat=inherit  Unit=inherit  AffineConversion=off
  Power Sensor (Three-Phase) : ee_lib/Sensors & Transducers/Power Sensor (Three-Phase)  load_type=ee.enum.passive.type_balanced.balanced  f0=60 Hz  config=ee.enum.with_neutral.no  rho=1
      settings: InternalSimscapePortConfiguration="{\"Bottom\":[],\"Left\":[{\"id\":\"N1\",\"label\":\"~1\",\"type\":\"foundation.electrical.three_phase\"}],\"Right\":[{\"id\":\"N2\",\"label\":\"~2\",\"type\":\"foundation.electrical.three_phase\"}],\"Top\":[{\"id\":\"Pm\",\"label\":\"P\",\"type\":\"output\"},{\"id\":\"Qm\",\"label\":\"Q\",\"type\":\"output\"}]}"
  Terminator : Terminator
  ~1 : PMIOPort  Side=Left
  ~2 : PMIOPort  Port=2  Side=Right
  wires:
  PS-Simulink Converter/1 -> Terminator/1  "P_Grid"
  connections:
  Power Sensor (Three-Phase)/LConn1 -- ~1/RConn1
  Power Sensor (Three-Phase)/RConn1 -- ~2/RConn1
  PS Terminator/LConn1 -- Power Sensor (Three-Phase)/LConn3
  PS-Simulink Converter/LConn1 -- Power Sensor (Three-Phase)/LConn2

== stateflow chart microgrid/URFC System/Operation mode controler ==
  state OFF
    during:
    I_EL = 0;
    I_FC = 0;
  state ON
    state FC_MODE
      during:
      I_EL = 0;
      I_FC = - I_ref;
    state EL_MODE
      during:
      I_EL = I_ref;
      I_FC = 0;
    (default) -> FC_MODE
    EL_MODE -> FC_MODE : [I_ref < 0]
    FC_MODE -> EL_MODE : [I_ref >  0]
  (default) -> OFF
  OFF -> ON : [I_ref ~= 0]
  ON -> OFF : [I_ref == 0]
  data: I_ref input; I_EL output; I_FC output
